simulink model "YJpto"  (R2025b)
settings: Solver=ode45  StartTime=0  StopTime=30  FixedStep=0.1  MaxStep=0.1  RelTol=1e-3  AbsTol=1e-3
settings Model: Creator=ndegoede  LastModifiedBy=ndegoede
settings SolverCC: AutoScaleAbsTol=off  DaesscMode=FullDebug  ZeroCrossControl=DisableAll  AutoInsertRateTranBlk=on  DecoupledContinuousIntegration=on
settings DataIOCC: ReturnWorkspaceOutputs=off
settings OptimizationCC: SimCompilerOptimization=on
settings SimscapeCC: SimscapeLogType=all  SimscapeLogOpenViewer=on

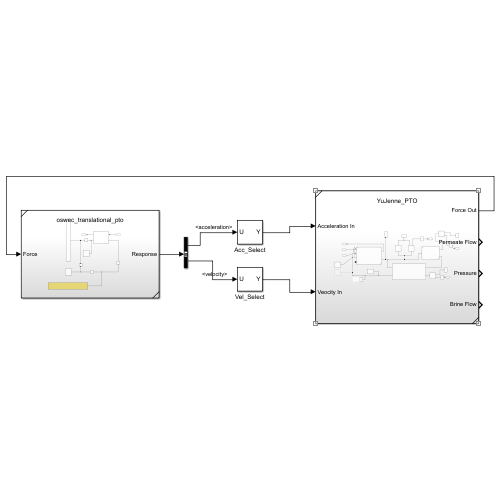
[thumbnail: Simulink's stored preview of the top-level diagram]
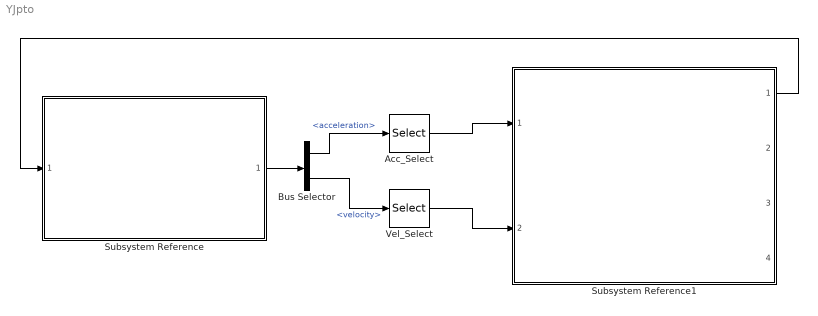
== system YJpto ==
  Acc_Select : Selector  InputPortWidth=6  IndexOptions=Index vector (dialog)  Indices=3  OutputSizes=1
  Bus Selector : BusSelector  OutputSignals=acceleration,velocity
  Subsystem Reference : Subsystem  ReferencedSubsystem=oswec_translational_pto
  Subsystem Reference1 : Subsystem  ReferencedSubsystem=YuJenne_PTO
  Vel_Select : Selector  InputPortWidth=6  IndexOptions=Index vector (dialog)  Indices=3  OutputSizes=1
  wires:
  Subsystem Reference/1 -> Bus Selector/1
  Bus Selector/2 -> Vel_Select/1  "<velocity>"
  Bus Selector/1 -> Acc_Select/1  "<acceleration>"
  Acc_Select/1 -> Subsystem Reference1/1
  Vel_Select/1 -> Subsystem Reference1/2
  Subsystem Reference1/1 -> Subsystem Reference/1
